simulink model "Codage_source"  (R2023b)
settings: Solver=VariableStepAuto  StartTime=0.0  StopTime=100000  RelTol=1e-3
undefined symbols (not defined in the file): graine, p1, Tb
settings Model: Creator=e2404931  LastModifiedBy=e2404931
settings DataIOCC: ReturnWorkspaceOutputs=off

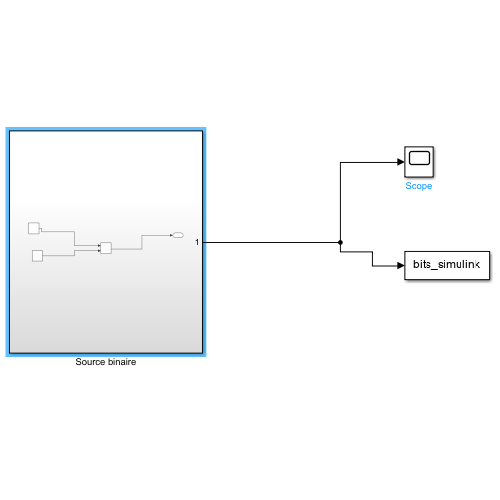
[thumbnail: Simulink's stored preview of the top-level diagram]
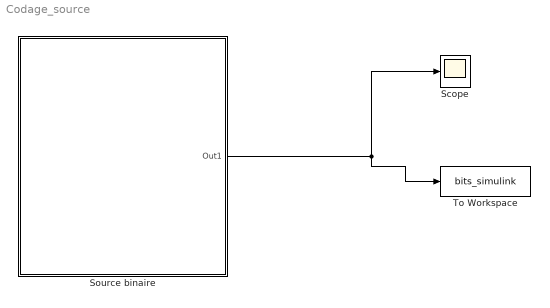
== system Codage_source ==
  Scope : Scope
  Source binaire : Subsystem
  To Workspace : ToWorkspace  VariableName=bits_simulink  SampleTime=-1
  wires:
  Source binaire/1(Out1) -> To Workspace/1, Scope/1

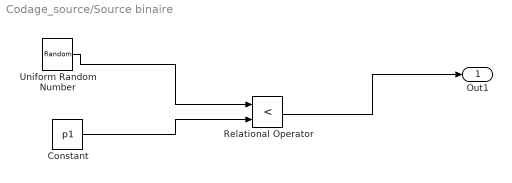
== system Codage_source/Source binaire ==
  Constant : Constant  Value=p1
  Relational Operator : RelationalOperator  Operator=<  OutDataTypeStr=boolean  RndMeth=Simplest  InputSameDT=off
  Uniform Random Number : UniformRandomNumber  Minimum=0  Seed=graine  SampleTime=Tb
  Out1 : Outport
  wires:
  Uniform Random Number/1 -> Relational Operator/1
  Constant/1 -> Relational Operator/2
  Relational Operator/1 -> Out1/1
